simulink model "KT_Robot_Pure_Pursuit"  (R2025b)
settings: Solver=FixedStepDiscrete  StartTime=0.0  StopTime=tEnd  FixedStep=Ts  RelTol=1e-3
model workspace (MAT data in the model file):
  Ts = 0.05
  initialPose = [0; -0.6; 0]
  pathData = [0  0  0  4; 4  0  4  3; 4  3  7  4; 8  3  11  3; 8  6  14  0]
  robot = [0.05; 0.3; 12; 2]
  settings = [0.55; 0.5; 0.05; 1; 1.308996939; 2; 0; 0.12; 0.05; 2400]
  tEnd = 120
settings Model: Creator=ADMIN  LastModifiedBy=ADMIN
settings DataIOCC: SaveOutput=off  SaveTime=off

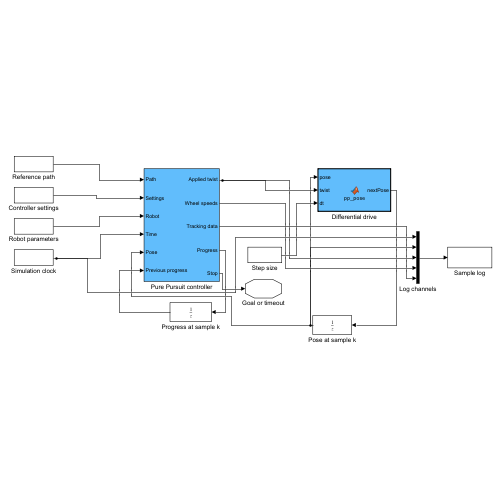
[thumbnail: Simulink's stored preview of the top-level diagram]
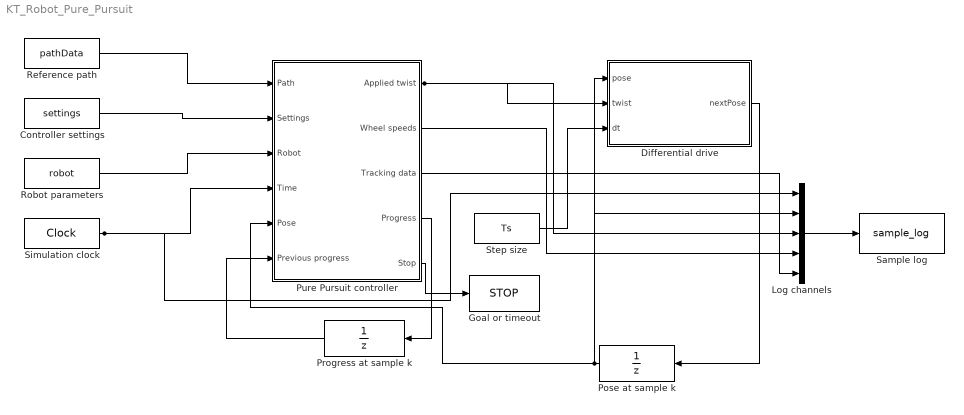
== system KT_Robot_Pure_Pursuit ==
  Controller settings : Constant  Value=settings
  Differential drive : MATLAB Function  TreatAsAtomicUnit=on
  Goal or timeout : Stop
  Log channels : Mux  Inputs=5
  Pose at sample k : UnitDelay  InitialCondition=initialPose  SampleTime=Ts  HasFrameUpgradeWarning=on
  Progress at sample k : UnitDelay  SampleTime=Ts  HasFrameUpgradeWarning=on
  Pure Pursuit controller : Subsystem
  Reference path : Constant  Value=pathData
  Robot parameters : Constant  Value=robot
  Sample log : ToWorkspace  VariableName=sample_log  SampleTime=-1
  Simulation clock : DigitalClock  SampleTime=Ts
  Step size : Constant  Value=Ts
  wires:
  Reference path/1 -> Pure Pursuit controller/1(Path)
  Controller settings/1 -> Pure Pursuit controller/2(Settings)
  Robot parameters/1 -> Pure Pursuit controller/3(Robot)
  Simulation clock/1 -> Pure Pursuit controller/4(Time), Log channels/1
  Pose at sample k/1 -> Pure Pursuit controller/5(Pose), Differential drive/1(pose), Log channels/2
  Progress at sample k/1 -> Pure Pursuit controller/6(Previous progress)
  Pure Pursuit controller/4(Progress) -> Progress at sample k/1
  Pure Pursuit controller/5(Stop) -> Goal or timeout/1
  Pure Pursuit controller/1(Applied twist) -> Differential drive/2(twist), Log channels/3
  Step size/1 -> Differential drive/3(dt)
  Differential drive/1(nextPose) -> Pose at sample k/1
  Pure Pursuit controller/2(Wheel speeds) -> Log channels/4
  Pure Pursuit controller/3(Tracking data) -> Log channels/5
  Log channels/1 -> Sample log/1

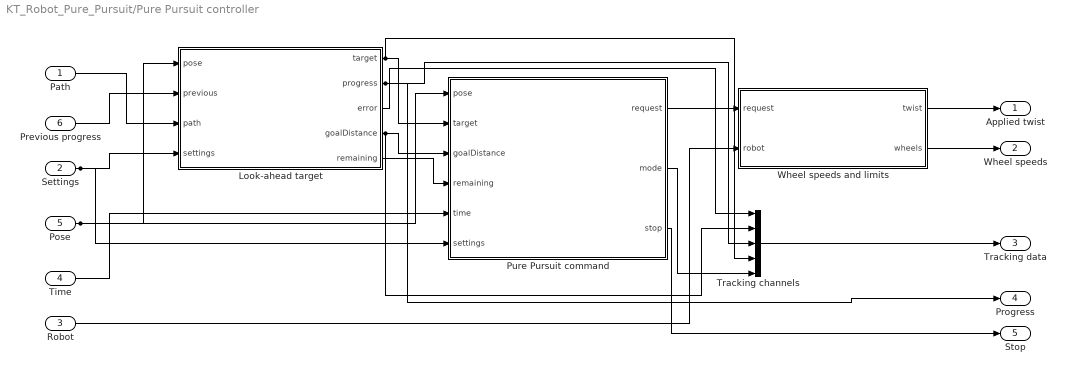
== system KT_Robot_Pure_Pursuit/Pure Pursuit controller ==
  Path : Inport
  Settings : Inport  Port=2
  Robot : Inport  Port=3
  Time : Inport  Port=4
  Pose : Inport  Port=5
  Previous progress : Inport  Port=6
  Look-ahead target : MATLAB Function  TreatAsAtomicUnit=on
  Pure Pursuit command : MATLAB Function  TreatAsAtomicUnit=on
  Tracking channels : Mux  Inputs=5
  Wheel speeds and limits : MATLAB Function  TreatAsAtomicUnit=on
  Applied twist : Outport
  Wheel speeds : Outport  Port=2
  Tracking data : Outport  Port=3
  Progress : Outport  Port=4
  Stop : Outport  Port=5
  wires:
  Pose/1 -> Look-ahead target/1(pose), Pure Pursuit command/1(pose)
  Previous progress/1 -> Look-ahead target/2(previous)
  Path/1 -> Look-ahead target/3(path)
  Settings/1 -> Look-ahead target/4(settings), Pure Pursuit command/6(settings)
  Look-ahead target/1(target) -> Pure Pursuit command/2(target), Tracking channels/4
  Look-ahead target/4(goalDistance) -> Pure Pursuit command/3(goalDistance), Tracking channels/2
  Look-ahead target/5(remaining) -> Pure Pursuit command/4(remaining)
  Time/1 -> Pure Pursuit command/5(time)
  Pure Pursuit command/1(request) -> Wheel speeds and limits/1(request)
  Robot/1 -> Wheel speeds and limits/2(robot)
  Wheel speeds and limits/1(twist) -> Applied twist/1
  Wheel speeds and limits/2(wheels) -> Wheel speeds/1
  Look-ahead target/3(error) -> Tracking channels/1
  Look-ahead target/2(progress) -> Tracking channels/3, Progress/1
  Pure Pursuit command/2(mode) -> Tracking channels/5
  Tracking channels/1 -> Tracking data/1
  Pure Pursuit command/3(stop) -> Stop/1

== matlab function KT_Robot_Pure_Pursuit/Pure Pursuit controller/Look-ahead target ==
  data: pose input; target output; previous input; path input; settings input; progress output; error output; goalDistance output; remaining output
function [target, progress, error, goalDistance, remaining] = pp_target(pose, previous, path, settings)
% Find the first forward circle intersection on the reference polyline.
xy = pose(1:2);
n = size(path,1);
total = path(n,3);
lookahead = settings(1);
progress = project(xy, path, previous, min(total, previous + max(2*lookahead,1)));
[~, error] = project(xy, path, 0, total);
goal = path(n,1:2).';
goalDistance = norm(goal - xy);
remaining = total - progress;
target = goal;
if remaining <= lookahead
    return
end

for i = 1:n-1
    if path(i+1,3) <= progress
        continue
    end
    p = path(i,1:2).';
    d = path(i+1,1:2).' - p;
    length = path(i,4);
    q = p - xy;
    a = dot(d,d);
    b = 2*dot(q,d);
    c = dot(q,q) - lookahead^2;
    disc = b*b - 4*a*c;
    if disc < 0
        continue
    end
    root = sqrt(disc);
    for u = [(-b-root)/(2*a), (-b+root)/(2*a)]
        if u >= 0 && u <= 1 && path(i,3) + u*length > progress + 1e-8
            target = p + u*d;
            return
        end
    end
end

s = min(progress + lookahead,total);
for i = 1:n-1
    if s < path(i+1,3) || i == n-1
        p = path(i,1:2).';
        d = path(i+1,1:2).' - p;
        target = p + ((s-path(i,3))/path(i,4))*d;
        return
    end
end
end

function [s, distance] = project(xy, path, first, last)
% Strict improvement preserves the first segment in a projection tie.
s = first;
distance = inf;
for i = 1:size(path,1)-1
    if path(i+1,3) < first || path(i,3) > last
        continue
    end
    p = path(i,1:2).';
    d = path(i+1,1:2).' - p;
    length = path(i,4);
    u = dot(xy-p,d)/length^2;
    low = max(0,(first-path(i,3))/length);
    high = min(1,(last-path(i,3))/length);
    u = min(max(u,low),high);
    e = norm(p + u*d - xy);
    if e < distance
        distance = e;
        s = path(i,3) + u*length;
    end
end
end

== matlab function KT_Robot_Pure_Pursuit/Differential drive ==
  data: pose input; nextPose output; twist input; dt input
function nextPose = pp_pose(pose,twist,dt)
% Exact motion under a zero-order-held command over one sample.
theta = pose(3);
v = twist(1);
omega = twist(2);
nextTheta = theta + omega*dt;
if abs(omega) < 1e-10
    displacement = v*[cos(theta);sin(theta)]*dt;
else
    displacement = (v/omega)*[sin(nextTheta)-sin(theta);cos(theta)-cos(nextTheta)];
end
nextPose = [pose(1:2) + displacement; mod(nextTheta+pi,2*pi)-pi];
end

== matlab function KT_Robot_Pure_Pursuit/Pure Pursuit controller/Pure Pursuit command ==
  data: pose input; request output; target input; goalDistance input; remaining input; time input; settings input; mode output; stop output
function [request, mode, stop] = pp_command(pose, target, goalDistance, remaining, time, settings)
% Modes: pursuit (0), alignment (1), goal (2), and timeout (3).
lookahead = settings(1);
nearEnd = remaining <= lookahead;
reached = nearEnd && goalDistance <= settings(3);
timeout = round(time/settings(9)) >= settings(10);
stop = reached || timeout;
request = zeros(2,1);
if stop
    mode = 3;
    if reached
        mode = 2;
    end
    return
end

offset = target - pose(1:2);
theta = pose(3);
alpha = mod(atan2(offset(2),offset(1)) - theta + pi,2*pi) - pi;
if abs(alpha) > settings(5)
    mode = 1;
    request(2) = settings(6)*alpha;
    return
end

mode = 0;
v = settings(2);
if nearEnd
    v = min(v,settings(4)*goalDistance);
end
yBody = -sin(theta)*offset(1) + cos(theta)*offset(2);
kappa = 2*yBody/max(dot(offset,offset),1e-12);
if settings(7) == 1
    v = min(v,sqrt(settings(8)/max(abs(kappa),1e-12)));
end
request = [v; v*kappa];
end

== matlab function KT_Robot_Pure_Pursuit/Pure Pursuit controller/Wheel speeds and limits ==
  data: request input; twist output; robot input; wheels output
function [twist,wheels] = pp_wheels(request, robot)
% Limit yaw first, then both wheels together to retain curvature.
radius = robot(1);
track = robot(2);
limited = request/max(1,abs(request(2))/robot(4));
v = limited(1);
omega = limited(2);
left = (v-track*omega/2)/radius;
right = (v+track*omega/2)/radius;
wheels = [left;right]/max([1,abs(left)/robot(3),abs(right)/robot(3)]);
twist = [radius*(wheels(1)+wheels(2))/2; radius*(wheels(2)-wheels(1))/track];
end
